simulink model "SOLUTION_04_Control_PID_and_HBridge"  (R2026b)
settings: Solver=ode15s  StopTime=10  MaxStep=0.01  AbsTol=1e-3  EnableMultiTasking=on
undefined symbols (not defined in the file or in its folder): my_DC_moto_OBJ, my_HBridge_OBJ, my_LINK_OBJ, X, Y, Z
libraries: fl_lib x9, sm_lib x8, nesl_utility x4, ee_lib x3, slpidlib x1, simulink x1
settings Model: Creator=bhorton  LastModifiedBy=bhorton
settings SolverCC: AutoScaleAbsTol=off
settings DataIOCC: LimitDataPoints=on  MaxDataPoints=10000
settings OptimizationCC: LifeSpan=inf  ReuseModelBlockBuffer=off
settings DebuggingCC: AllowSymbolicDim=off  ArithmeticOperatorsInVariantConditions=warning  SFExecutionAtInitializationDiag=none  SFNoUnconditionalDefaultTransitionDiag=warning  SFUnexpectedBacktrackingDiag=warning  SubsystemReferenceDiagnosticForUnitTest=warning
settings SFSimCC: CustomCodeUndefinedFunction=UseInterfaceOnly  SimUseLocalCustomCode=off
settings RTWCC: DLArmComputeVersion=19.05  RTWUseLocalCustomCode=off
settings CodeAppCC: StateflowObjectComments=on
settings GRTTargetCC: TargetLangStandard=C89/C90 (ANSI)
settings ConfigComp: CovExternalEMLEnable=off  CovSFcnEnable=off  CovSaveCumulativeToWorkspaceVar=on  CovSaveSingleToWorkspaceVar=on
settings SimscapeCC: SimscapeLogType=all  SimscapeUseEnergyAccounting=off
settings ExplorerConfigSet: InternalSimMechanicsExplorerSettings=|
  | <ExplorerConfiguration>
  | 
  |   <canonicalview>default</canonicalview>
  | 
  |   <TilePanel>
  |     <TileInfo>
  |       <Tiles Columns="2" Count="3" Height="706" Rows="2" Width="1078">
  |         <Row Weight="0.500709"/>
  |         <Row Weight="0.499291"/>
  |         <Column Weight="0.500464"/>
  |         <Column Weight="0.499536"/>
  |         <Tile Height="2" Width="1" X="0" Y="0"/>
  |         <Tile Height="1" Width="1" X="1" Y="0"/>
  |         <Tile Height="1" Width="1" X="1" Y="1"/>
  |       </Tiles>
  |     </TileInfo>
  |     <SceneInfo>
  |       <SceneViewer>
  |         <IsThisViewStd>
  |           <IsStandardView>off</IsStandardView>
  |           <StandardViewName>Front</StandardViewName>
  |         </IsThisViewStd>
  |         <BGColor>
  |           <R>1</R>
  |           <G>1</G>
  |           <B>1</B>
  |           <A>1</A>
  |         </BGColor>
  |         <Camera>
  |           <DoPerspective>off</DoPerspective>
  |           <Position>
  |             <X>0.74892143739918005</X>
  |             <Y>-0.62784979879609726</Y>
  |             <Z>0.69336876380477952</Z>
  |           </Position>
  |           <Center>
  |             <X>0.053221437399180033</X>
  |             <Y>0.067850201203902699</Y>
  |             <Z>-0.0023312361952205086</Z>
  |           </Center>
  |           <Up>
  |             <X>-0.40824829046386307</X>
  |             <Y>0.40824829046386307</Y>
  |             <Z>0.81649658092772615</Z>
  |           </Up>
  |           <XLim>0.18530968569291589</XLim>
  |           <YLim>0.18530968569291589</YLim>
  |           <ViewLimDist>0.01</ViewLimDist>
  |         </Camera>
  |       </SceneViewer>
  |       <SceneViewer>
  |         <IsThisViewStd>
  |           <IsStandardView>off</IsStandardView>
  |           <StandardViewName>Front</StandardViewName>
  |         </IsThisViewStd>
  |         <BGColor>
  |           <R>1</R>
  |           <G>1</G>
  |           <B>1</B>
  |           <A>1</A>
  |         </BGColor>
  |         <Camera>
  |           <DoPerspective>off</DoPerspective>
  |           <Position>
  |             <X>0.024441165727511753</X>
  |             <Y>0.15035032949724758</Y>
  |             <Z>1.8651286729311369</Z>
  |           </Position>
  |           <Center>
  |             <X>0.024441165727511753</X>
  |             <Y>0.15035032949724758</Y>
  |             <Z>0.14374999981373549</Z>
  |           </Center>
  |           <Up>
  |             <X>-1</X>
  |             <Y>-1.8735013540549517e-16</Y>
  |             <Z>0</Z>
  |           </Up>
  |           <XLim>0.15951004814416869</XLim>
  |           <YLim>0.15951004814416869</YLim>
  |           <ViewLimDist>0.01</ViewLimDist>
  |         </Camera>
  |       </SceneViewer>
  |       <SceneViewer>
  |         <IsThisViewStd>
  |           <IsStandardView>off</IsStandardView>
  |           <StandardViewName>Front</StandardViewName>
  |         </IsThisViewStd>
  |         <BGColor>
  |           <R>1</R>
  |           <G>1</G>
  |           <B>1</B>
  |           <A>1</A>
  |         </BGColor>
  |         <Camera>
  |           <DoPerspective>off</DoPerspective>
  |           <Position>
  |             <X>1.4204228299283366</X>
  |             <Y>0.16790494784880997</Y>
  |             <Z>-0.11689190590831854</Z>
  |           </Position>
  |           <Center>
  |             <X>0.096938775434177712</X>
  |             <Y>0.16790494784880997</Y>
  |             <Z>-0.11689190590831854</Z>
  |           </Center>
  |           <Up>
  |             <X>0</X>
  |             <Y>0</Y>
  |             <Z>1</Z>
  |           </Up>
  |           <XLim>0.20515932592869371</XLim>
  |           <YLim>0.20515932592869371</YLim>
  |           <ViewLimDist>0.01</ViewLimDist>
  |         </Camera>
  |       </SceneViewer>
  |     </SceneInfo>
  |   </TilePanel>
  | 
  |   <MechEditorPanel>
  |     <GfxPanelCameraMap/>
  |     <Cameras/>
  |     <VideoCreator>
  |       <IncludeTiles>All</IncludeTiles>
  |       <IncludeTime>on</IncludeTime>
  |       <IncludeWorldFrame>off</IncludeWorldFrame>
  |       <PlaybackSpeedRatio>1</PlaybackSpeedRatio>
  |       <FrameRate>30</FrameRate>
  |       <FrameSize>auto</FrameSize>
  |       <VideoFormat>UncompressedAVI</VideoFormat>
  |     </VideoCreator>
  |   </MechEditorPanel>
  | 
  |   <PlaybackSettings>
  |     <PlaybackSpeedFactor>1</PlaybackSpeedFactor>
  |   </PlaybackSettings>
  | 
  | </ExplorerConfiguration>

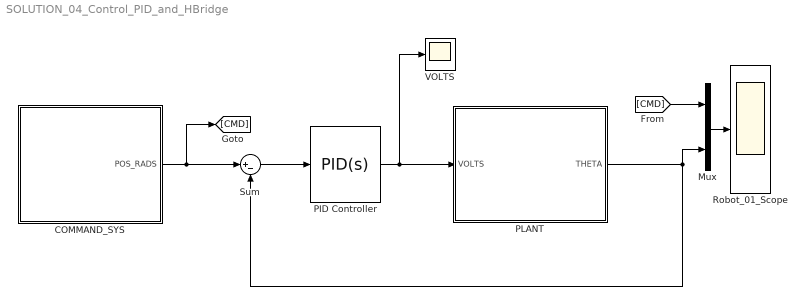
== system SOLUTION_04_Control_PID_and_HBridge ==
  COMMAND_SYS : Subsystem
  Mux : Mux  Inputs=2
  PID Controller : slpidlib/PID Controller  Controller=PID  Form=Parallel  TimeDomain=Continuous-time  UseExternalTs=off  SampleTime=-1  IntegratorMethod=Forward Euler  FilterMethod=Forward Euler  ControllerParametersSource=internal  P=21.8439839664318  I=71.2671260044186  UseKiTs=off  D=1.50425908128224  UseExternalDerivativeSource=off  N=168.946400688862  UseFilter=on  TunerSelectOption=Transfer Function Based (PID Tuner App)  InitialConditionSource=internal  InitialConditionForIntegrator=0  InitialConditionForFilter=0  DifferentiatorICPrevScaledInput=0  ExternalReset=none  TrackingMode=off  Kt=1  LimitOutput=off  SatLimitsSource=internal  UpperSaturationLimit=inf  LowerSaturationLimit=-inf  LinearizeAsGain=on  AntiWindupMode=none  Kb=1  LimitIntegrator=off  UpperIntegratorSaturationLimit=inf  LowerIntegratorSaturationLimit=-inf  POutMin=[]  POutMax=[]  IOutMin=[]  IOutMax=[]  DOutMin=[]  DOutMax=[]  NOutMin=[]  NOutMax=[]  SumOutMin=[]  SumOutMax=[]  SaturationOutMin=[]  SaturationOutMax=[]  PParamMin=[]  PParamMax=[]  IParamMin=[]  IParamMax=[]  DParamMin=[]  DParamMax=[]  NParamMin=[]  NParamMax=[]  KbParamMin=[]  KbParamMax=[]  KtParamMin=[]  KtParamMax=[]  KbOutMin=[]  KbOutMax=[]  KtOutMin=[]  KtOutMax=[]  IntegratorOutMin=[]  IntegratorOutMax=[]  FilterOutMin=[]  FilterOutMax=[]  SumI1OutMin=[]  SumI1OutMax=[]  SumI2OutMin=[]  SumI2OutMax=[]  SumI3OutMin=[]  SumI3OutMax=[]  SumI4OutMin=[]  SumI4OutMax=[]  SumDOutMin=[]  SumDOutMax=[]  DifferentiatorOutMin=[]  DifferentiatorOutMax=[]  FilterDiffOutCoefMin=[]  FilterDiffOutCoefMax=[]  ReciprocalOutMin=[]  ReciprocalOutMax=[]  SumDenOutMin=[]  SumDenOutMax=[]  SumNumOutMin=[]  SumNumOutMax=[]  DivideOutMin=[]  DivideOutMax=[]  UdiffTsProdOutMin=[]  UdiffTsProdOutMax=[]  NTsProdOutMin=[]  NTsProdOutMax=[]  UintegralTsProdOutMin=[]  UintegralTsProdOutMax=[]  UngainTsProdOutMin=[]  UngainTsProdOutMax=[]  ClampingZeroOutDataTypeStr=Inherit: Inherit via back propagation  ClampingZeroOutMin=[]  ClampingZeroOutMax=[]  FilterDenConstantOutDataTypeStr=Inherit: Inherit via back propagation  FilterDenConstantOutMin=[]  FilterDenConstantOutMax=[]  PCopyOutDataTypeStr=Inherit: Inherit via back propagation  PCopyOutMin=[]  PCopyOutMax=[]  NCopyOutDataTypeStr=Inherit: Inherit via back propagation  NCopyOutMin=[]  NCopyOutMax=[]  IntegratorContinuousStateAttributes=''  IntegratorStateMustResolveToSignalObject=off  IntegratorRTWStateStorageClass=Auto  FilterContinuousStateAttributes=''  FilterStateMustResolveToSignalObject=off  FilterRTWStateStorageClass=Auto  ParallelPVariant=InternalParameters  IdealPVariant=Disabled  IVariant=InternalParameters  DVariant=InternalParameters  IntegratorVariant=Continuous  SatVariant=Disabled  AWVariant=Passthrough  PCopyVariant=Disabled  TRVariant=Disabled  FdbkBlocksVariant=Forward  IdealPFdbkVariant=Disabled  SatFdbkVariant=Disabled  DerivativeFilterVariant=ContFilter  NVariant=InternalParameters  NCopyVariant=Disabled  FilterICVariant=InternalICsFilter  IntegratorICVariant=InternalICs  ExternalResetVariant=Disabled  TRSumVariant=Passthrough  SumFdbkVariant=Disabled  SumVariant=Sum_PID  TsampFilterVariant=InternalTs  TsampNgainVariant=Passthrough  TsampIntegralVariant=Disabled_SignalSpec  ExternalSaturationOutDataTypeStr=Inherit: Same as second input  DerivativeSourceVariant=ErrorSignal  PreIntVariant=InternalPreInt
  PLANT : Subsystem
  Robot_01_Scope : Scope
      settings: ActiveDisplayYMinimum=-0.1366602346180848  ActiveDisplayYMaximum=0.954029318573031
  Sum : Sum  Inputs=|+-
  VOLTS : Scope
      settings: ActiveDisplayYMinimum=-3.0831786783905404  ActiveDisplayYMaximum=21.688685222638515  DataLoggingVariableName=ScopeData2
  wires:
  Sum/1 -> PID Controller/1
  PID Controller/1 -> PLANT/1(VOLTS), VOLTS/1
  [CMD] -> Mux/1
  Mux/1 -> Robot_01_Scope/1
  PLANT/1(THETA) -> Sum/2, Mux/2
  COMMAND_SYS/1(POS_RADS) -> [CMD], Sum/1

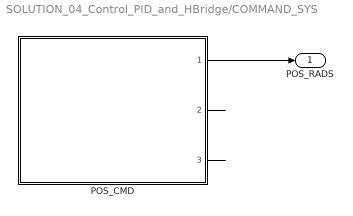
== system SOLUTION_04_Control_PID_and_HBridge/COMMAND_SYS ==
  POS_CMD : Subsystem  ReferencedSubsystem=COMPONENT_POS_CMD
  POS_RADS : Outport
  wires:
  POS_CMD/1 -> POS_RADS/1
  POS_CMD/2 -> ?
  POS_CMD/3 -> ?

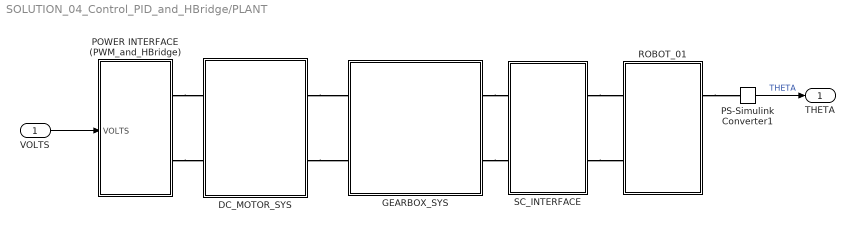
== system SOLUTION_04_Control_PID_and_HBridge/PLANT ==
  VOLTS : Inport
  DC_MOTOR_SYS : Subsystem
  GEARBOX_SYS : Subsystem
  POWER INTERFACE (PWM_and_HBridge) : Subsystem
  PS-Simulink Converter1 : nesl_utility/PS-Simulink Converter  PhysicalDomain=network_engine_domain  SubClassName=ps_output  LeftPortType=input  RightPortType=output  PseudoPeriodic=off  Frequencies=[]  VectorFormat=inherit  Unit=rad  AffineConversion=off
      settings: AttributesFormatString=UNITS= (%<Unit>)
  ROBOT_01 : Subsystem
  SC_INTERFACE : Subsystem
  THETA : Outport
  wires:
  VOLTS/1 -> POWER INTERFACE (PWM_and_HBridge)/1(VOLTS)
  PS-Simulink Converter1/1 -> THETA/1  "THETA"
  connections:
  DC_MOTOR_SYS/RConn1 -- GEARBOX_SYS/LConn1
  SC_INTERFACE/RConn2 -- ROBOT_01/LConn2
  POWER INTERFACE (PWM_and_HBridge)/RConn2 -- DC_MOTOR_SYS/LConn2
  POWER INTERFACE (PWM_and_HBridge)/RConn1 -- DC_MOTOR_SYS/LConn1
  GEARBOX_SYS/RConn2 -- SC_INTERFACE/LConn2
  GEARBOX_SYS/RConn1 -- SC_INTERFACE/LConn1
  SC_INTERFACE/RConn1 -- ROBOT_01/LConn1
  ROBOT_01/RConn1 -- PS-Simulink Converter1/LConn1
  DC_MOTOR_SYS/RConn2 -- GEARBOX_SYS/LConn2

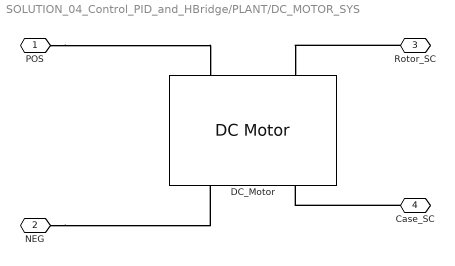
== system SOLUTION_04_Control_PID_and_HBridge/PLANT/DC_MOTOR_SYS ==
  DC_Motor : ee_lib/Electromechanical/Brushed Motors/DC Motor  field_option=ee.enum.field_option.pm  Rf=100 Ohm  Lf=1 H  Laf=0.15 H  If0=0 A  parameterization=ee.enum.dcparam_option.circuit_param  Ra=my_DC_moto_OBJ.arm_R Ohm  La=my_DC_moto_OBJ.arm_L H  emf_or_torque=ee.enum.emf_or_torque.ki  Kv=0.072e-3 V/rpm  Ki=my_DC_moto_OBJ.K_t N*m/A  T_stall=0.24e-3 N*m  w_max=19100 rpm  w_rated=15000 rpm  P_rated=0.08 W  V_rated=1.5 V  lam_param=ee.enum.lam_param.damping  i_noload=0 A  V_i_noload=1.5 V  J=my_DC_moto_OBJ.rotor_I kg*m^2  lam=my_DC_moto_OBJ.rotor_damp N*m*s/rad  speed0=0 rpm  alpha=3.93e-3 1/K  Tmeas=25 degC  thermal_mass=100 J/K  initial_temperature=25 degC
  POS : PMIOPort  Side=Left
  NEG : PMIOPort  Port=2  Side=Left
  Rotor_SC : PMIOPort  Port=3  Side=Right
  Case_SC : PMIOPort  Port=4  Side=Right
  connections:
  NEG/RConn1 -- DC_Motor/RConn1
  POS/RConn1 -- DC_Motor/LConn1
  Rotor_SC/RConn1 -- DC_Motor/LConn2
  Case_SC/RConn1 -- DC_Motor/RConn2

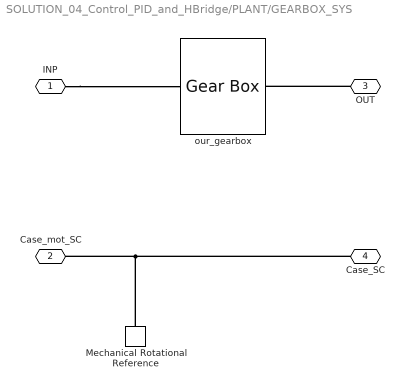
== system SOLUTION_04_Control_PID_and_HBridge/PLANT/GEARBOX_SYS ==
  Mechanical Rotational Reference : fl_lib/Mechanical/Rotational Elements/Mechanical Rotational Reference
  our_gearbox : fl_lib/Mechanical/Mechanisms/Gear Box  ratio=my_gbox_OBJ.N_gear  t_in_specify=off  t_in_priority=None  t_in=0 N*m  t_in_nominal_specify=off  t_in_nominal_value=1  t_in_nominal_unit=N*m  t_out_specify=off  t_out_priority=None  t_out=0 N*m  t_out_nominal_specify=off  t_out_nominal_value=1  t_out_nominal_unit=N*m
      settings: AttributesFormatString=N = w_IN / w_OUT = %<ratio>
  INP : PMIOPort  Side=Left
  Case_mot_SC : PMIOPort  Port=2  Side=Left
  OUT : PMIOPort  Port=3  Side=Right
  Case_SC : PMIOPort  Port=4  Side=Right
  connections:
  Mechanical Rotational Reference/LConn1 -- Case_mot_SC/RConn1 -- Case_SC/RConn1
  INP/RConn1 -- our_gearbox/LConn1
  OUT/RConn1 -- our_gearbox/RConn1

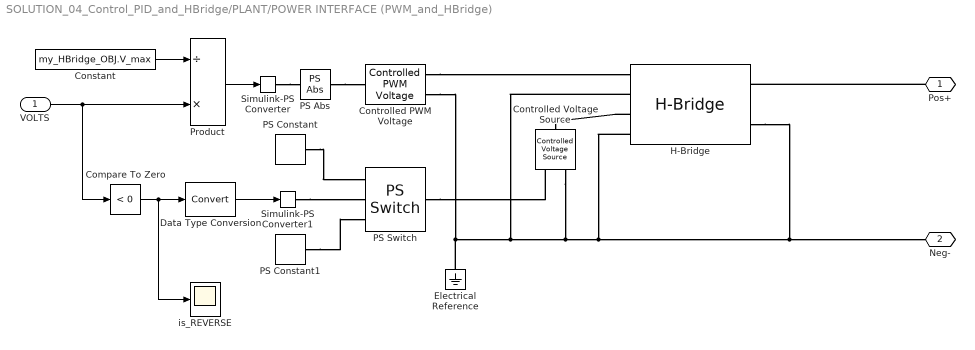
== system SOLUTION_04_Control_PID_and_HBridge/PLANT/POWER INTERFACE (PWM_and_HBridge) ==
  VOLTS : Inport
  Compare To Zero : simulink/Logic and Bit Operations/Compare To Zero  relop=<  OutDataTypeStr=uint8
  Constant : Constant  Value=my_HBridge_OBJ.V_max
  Controlled PWM Voltage : ee_lib/Integrated Circuits/Controlled PWM Voltage  F=80 kHz  TD=0 s  pulse_width_offset=0 s  pulse_min=0 s  pwm_or_av=ee.enum.pwm_or_av.averaged  event_type=ee.enum.ic.event.asynchronous  sample_time=1e-6 s  Vmin=0 V  Vmax=24 V  Vm=my_HBridge_OBJ.V_max V  u_min=0  u_max=1
  Controlled Voltage Source : fl_lib/Electrical/Electrical Sources/Controlled Voltage Source
  Data Type Conversion : DataTypeConversion  SaturateOnIntegerOverflow=off  RndMeth=Floor
  Electrical Reference : fl_lib/Electrical/Electrical Elements/Electrical Reference
  H-Bridge : ee_lib/Semiconductors & Converters/Converters/H-Bridge  supply_ports=ee.enum.supply_ports.hidesupply  pwm_or_av=ee.enum.pwm_or_av.averaged  discontinuous=ee.enum.current_profile.continuous  freewheeling_mode=ee.enum.converters.freewheeling_mode.one_switch_one_diode  Rload=10 Ohm  Lload=1e-5 H  F=10 kHz  regenerative_braking_mode=ee.enum.converters.regenerative_braking_mode.always_enabled  Venable=0.1 V  Vmax=my_HBridge_OBJ.V_max V  Vreverse=2.5 V  Vbrake=2.5 V  Vm=my_HBridge_OBJ.V_max V  Ron=my_HBridge_OBJ.R Ohm  Don=my_HBridge_OBJ.R_diode Ohm  Goff=1e-6 S  Tmeas=298.15 K  Ron2=0.1 Ohm  Don2=0.05 Ohm  Tmeas2=398.15 K  thermal_mass=100 J/K  initial_temperature=298.15 K
  PS Abs : fl_lib/Physical Signals/Nonlinear Operators/PS Abs  ZeroCross=true
  PS Constant : fl_lib/Physical Signals/Sources/PS Constant  constant=5 V
  PS Constant1 : fl_lib/Physical Signals/Sources/PS Constant  constant=0 V
  PS Switch : fl_lib/Physical Signals/Nonlinear Operators/PS Switch  Threshold=0.5  ZeroCross=true
  Product : Product  Inputs=/*
  Simulink-PS Converter : nesl_utility/Simulink-PS Converter  PhysicalDomain=network_engine_domain  SubClassName=ps_input  LeftPortType=input  RightPortType=output  PseudoPeriodic=off  Frequencies=[]  NoiseDistribution=none  NoiseParameters=[]  Unit=1  AffineConversion=off  FilteringAndDerivatives=provide  SimscapeFilterOrder=1  InputFilterTimeConstant=0.001  UdotUserProvided=0
  Simulink-PS Converter1 : nesl_utility/Simulink-PS Converter  PhysicalDomain=network_engine_domain  SubClassName=ps_input  LeftPortType=input  RightPortType=output  PseudoPeriodic=off  Frequencies=[]  NoiseDistribution=none  NoiseParameters=[]  Unit=1  AffineConversion=off  FilteringAndDerivatives=provide  SimscapeFilterOrder=1  InputFilterTimeConstant=0.001  UdotUserProvided=0
  is_REVERSE : Scope
      settings: ActiveDisplayYMinimum=-0.21102162286492421  ActiveDisplayYMaximum=1.2157883377749992  DataLoggingVariableName=ScopeData2
  Pos+ : PMIOPort  Side=Right
  Neg- : PMIOPort  Port=2  Side=Right
  wires:
  VOLTS/1 -> Product/2, Compare To Zero/1
  Data Type Conversion/1 -> Simulink-PS Converter1/1
  Compare To Zero/1 -> is_REVERSE/1, Data Type Conversion/1
  Product/1 -> Simulink-PS Converter/1
  Constant/1 -> Product/1
  connections:
  Pos+/RConn1 -- H-Bridge/RConn1
  Controlled PWM Voltage/RConn1 -- H-Bridge/LConn1
  Controlled PWM Voltage/RConn2 -- Electrical Reference/LConn1 -- H-Bridge/LConn2 -- Controlled Voltage Source/RConn2 -- H-Bridge/LConn4 -- H-Bridge/RConn2 -- Neg-/RConn1
  PS Switch/RConn1 -- Controlled Voltage Source/RConn1
  PS Abs/RConn1 -- Controlled PWM Voltage/LConn1
  PS Constant/RConn1 -- PS Switch/LConn1
  PS Constant1/RConn1 -- PS Switch/LConn3
  Simulink-PS Converter/RConn1 -- PS Abs/LConn1
  H-Bridge/LConn3 -- Controlled Voltage Source/LConn1
  Simulink-PS Converter1/RConn1 -- PS Switch/LConn2

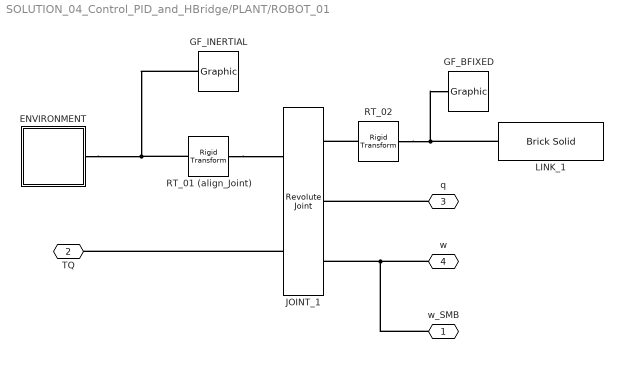
== system SOLUTION_04_Control_PID_and_HBridge/PLANT/ROBOT_01 ==
  ENVIRONMENT : Subsystem
  GF_BFIXED : sm_lib/Body Elements/Graphic  GraphicType=Marker  MarkerShape=Frame  MarkerSize=50  GraphicVisPropType=SimpleVisualProperties  GraphicDiffuseColor=[0.6667 0.6667 1]  GraphicOpacity=1  GraphicSpecularColor=[0.5 0.5 0.5 1.0]  GraphicAmbientColor=[0.15 0.15 0.15 1.0]  GraphicEmissiveColor=[0.0 0.0 0.0 1.0]  GraphicShininess=75
  GF_INERTIAL : sm_lib/Body Elements/Graphic  GraphicType=Marker  MarkerShape=Frame  MarkerSize=55  GraphicVisPropType=SimpleVisualProperties  GraphicDiffuseColor=[1 0 0]  GraphicOpacity=1  GraphicSpecularColor=[0.5 0.5 0.5 1.0]  GraphicAmbientColor=[0.15 0.15 0.15 1.0]  GraphicEmissiveColor=[0.0 0.0 0.0 1.0]  GraphicShininess=75
  JOINT_1 : sm_lib/Joints/Revolute Joint  JointMode=Normal  CompositeWrenchDir=FollowerOnBase  CompositeWrenchFrame=BaseFrame  SenseConstraintForce=off  SenseConstraintTorque=off  SenseTotalForce=off  SenseTotalTorque=off  PositionTargetSpecify=on  PositionTargetPriority=High  PositionTargetValue=my_joint_1_OBJ.theta  PositionTargetValueUnits=rad  VelocityTargetSpecify=on  VelocityTargetPriority=High  VelocityTargetValue=my_joint_1_OBJ.theta_dot  VelocityTargetValueUnits=rad/s  EquilibriumPosition=0  EquilibriumPositionUnits=deg  SpringStiffness=0  SpringStiffnessUnits=N*m/deg  DampingCoefficient=my_joint_1_OBJ.Damp  DampingCoefficientUnits=N*m*s/rad  LowerLimitSpecify=off  LowerLimitBound=-90  LowerLimitBoundUnits=deg  LowerLimitStiffness=1e4  LowerLimitStiffnessUnits=N*m/deg  LowerLimitDamping=10  LowerLimitDampingUnits=N*m/(deg/s)  LowerLimitTransitionRegionWidth=0.1  LowerLimitTransitionRegionWidthUnits=deg  UpperLimitSpecify=off  UpperLimitBound=90  UpperLimitBoundUnits=deg  UpperLimitStiffness=1e4  UpperLimitStiffnessUnits=N*m/deg  UpperLimitDamping=10  UpperLimitDampingUnits=N*m/(deg/s)  UpperLimitTransitionRegionWidth=0.1  UpperLimitTransitionRegionWidthUnits=deg  TorqueActuationMode=InputTorque  MotionActuationMode=ComputedMotion  SensePosition=on  SenseVelocity=on  SenseAcceleration=off  SenseTorqueForce=off  SenseLowerLimitTorqueForce=off  SenseUpperLimitTorqueForce=off
  LINK_1 : sm_lib/Body Elements/Brick Solid  BrickDimensions=my_LINK_OBJ.vec_XYZ  BrickDimensionsUnits=m  ExportEntireGeometry=off  InertiaType=CalculateFromGeometry  BasedOnType=Mass  Density=1000  DensityUnits=kg/m^3  Mass=my_LINK_OBJ.Mass  MassUnits=kg  CenterOfMass=[0 0 0]  CenterOfMassUnits=m  MomentsOfInertia=[1 1 1]  MomentsOfInertiaUnits=kg*m^2  ProductsOfInertia=[0 0 0]  ProductsOfInertiaUnits=kg*m^2  GraphicType=FromGeometry  MarkerShape=Sphere  MarkerSize=10  GraphicVisPropType=SimpleVisualProperties  GraphicDiffuseColor=[0 0.6667 1]  GraphicOpacity=1.0  GraphicSpecularColor=[0.5 0.5 0.5 1.0]  GraphicAmbientColor=[0.15 0.15 0.15 1.0]  GraphicEmissiveColor=[0.0 0.0 0.0 1.0]  GraphicShininess=75  DoExposeReferenceFrame=on  SerializedFrames=|
      | <Frames>
      | 
      |   <Frame>
      |     <Id>Frame1</Id>
      |     <Value>
      |       <Name>LEFT</Name>
      |       <Origin>
      |         <Source>GeometricFeature</Source>
      |         <FeatureName>-y surface</FeatureName>
      |       </Origin>
      |       <PrimaryAxis>
      |         <DefinedDirection>+Z</DefinedDirection>
      |         <Source>ReferenceFrame</Source>
      |         <SourceDirection>+Z</SourceDirection>
      |         <FeatureName></FeatureName>
      |       </PrimaryAxis>
      |       <SecondaryAxis>
      |         <DefinedDirection>+X</DefinedDirection>
      |         <Source>ReferenceFrame</Source>
      |         <SourceDirection>+X</SourceDirection>
      |         <FeatureName></FeatureName>
      |       </SecondaryAxis>
      |     </Value>
      |   </Frame>
      | 
      | </Frames>
  RT_01 (align_Joint) : sm_lib/Frames and Transforms/Rigid Transform  RotationMethod=StandardAxis  FollAlignAxisA=+Z  BaseAlignAxisA=+X  FollAlignAxisB=+Y  BaseAlignAxisB=+Y  RotationStandardAxis=+Y  RotationAngle=90  RotationAngleUnits=deg  RotationArbitraryAxis=[0 0 1]  RotationSequenceAxes=FollowerAxes  RotationSequence=XYX  RotationSequenceAngles=[0 0 0]  RotationSequenceAnglesUnits=deg  RotationMatrix=[1 0 0;0 1 0;0 0 1]  Quaternion=[1 0 0 0]  TranslationMethod=None  TranslationCartesianOffset=[0 0 0]  TranslationCartesianOffsetUnits=m  TranslationStandardAxis=+Z  TranslationStandardOffset=0  TranslationStandardOffsetUnits=m  TranslationROffset=0  TranslationROffsetUnits=m  TranslationThetaOffset=0  TranslationThetaOffsetUnits=deg  TranslationZOffset=0  TranslationZOffsetUnits=m
  RT_02 : sm_lib/Frames and Transforms/Rigid Transform  RotationMethod=StandardAxis  FollAlignAxisA=+X  BaseAlignAxisA=+Z  FollAlignAxisB=+Y  BaseAlignAxisB=+Y  RotationStandardAxis=+Y  RotationAngle=-90  RotationAngleUnits=deg  RotationArbitraryAxis=[0 0 1]  RotationSequenceAxes=FollowerAxes  RotationSequence=XYX  RotationSequenceAngles=[0 0 0]  RotationSequenceAnglesUnits=deg  RotationMatrix=[1 0 0;0 1 0;0 0 1]  Quaternion=[1 0 0 0]  TranslationMethod=None  TranslationCartesianOffset=[0 0 0]  TranslationCartesianOffsetUnits=m  TranslationStandardAxis=+Z  TranslationStandardOffset=0  TranslationStandardOffsetUnits=m  TranslationROffset=0  TranslationROffsetUnits=m  TranslationThetaOffset=0  TranslationThetaOffsetUnits=deg  TranslationZOffset=0  TranslationZOffsetUnits=m
  w_SMB : PMIOPort  Side=Left
  TQ : PMIOPort  Port=2  Side=Left
  q : PMIOPort  Port=3  Side=Right
  w : PMIOPort  Port=4  Side=Right
  connections:
  RT_02/RConn1 -- LINK_1/LConn1 -- GF_BFIXED/RConn1
  GF_INERTIAL/RConn1 -- ENVIRONMENT/RConn1 -- RT_01 (align_Joint)/LConn1
  RT_01 (align_Joint)/RConn1 -- JOINT_1/LConn1
  RT_02/LConn1 -- JOINT_1/RConn1
  q/RConn1 -- JOINT_1/RConn2
  w/RConn1 -- w_SMB/RConn1 -- JOINT_1/RConn3
  JOINT_1/LConn2 -- TQ/RConn1

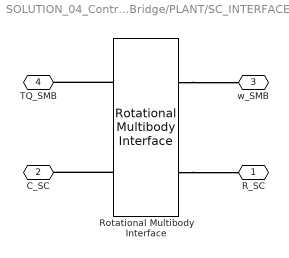
== system SOLUTION_04_Control_PID_and_HBridge/PLANT/SC_INTERFACE ==
  Rotational Multibody Interface : fl_lib/Mechanical/Multibody Interfaces/Rotational Multibody Interface
  R_SC : PMIOPort  Side=Left
  C_SC : PMIOPort  Port=2  Side=Left
  w_SMB : PMIOPort  Port=3  Side=Right
  TQ_SMB : PMIOPort  Port=4  Side=Right
  connections:
  Rotational Multibody Interface/LConn1 -- TQ_SMB/RConn1
  Rotational Multibody Interface/LConn2 -- C_SC/RConn1
  Rotational Multibody Interface/RConn1 -- w_SMB/RConn1
  Rotational Multibody Interface/RConn2 -- R_SC/RConn1

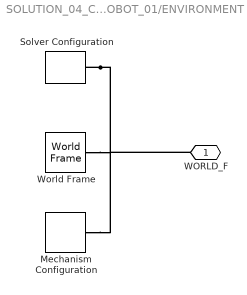
== system SOLUTION_04_Control_PID_and_HBridge/PLANT/ROBOT_01/ENVIRONMENT ==
  Mechanism Configuration : sm_lib/Utilities/Mechanism Configuration  UniformGravity=Constant  GravityVector=gravity_vec  GravityVectorUnits=m/s^2  LinearizationDelta=0.001  JointModeTransitionNonlinearIterations=2
  Solver Configuration : nesl_utility/Solver Configuration  PhysicalDomain=network_engine_domain  SubClassName=solver  LeftPortType=input  RightPortType=generic  Tones=[]  Harmonics=[]  SimulateNoise=off  Profile=off  UseLocalSampling=off  EnableSwitchedLinearOptims=on  FrequencyDomain=off  UseCCode=off  RelTol=0.001  AbsTol=1e-06  MinStep=1e-09  ToWorkspace=off  RevertToSquareIcSolve=off  NumHomotopyIterations=100  PhasorMode=off  PhasorModeNumHarmonics=1  ConsistencySolver=NEWTON_XTOL_AFTER_FTOL  CanonicalOrdering=UNORDERED  OptimizeIntermediates=UNOPTIMIZED  MulticoreSolverChoice=BACKWARD_EULER  IndexReductionMethod=DerivativeReplacement  DoDC=off  ResidualTolerance=1e-09  ConsistencyTolSource=GLOBAL  ConsistencyAbsTol=0.001  ConsistencyRelTol=0.001  ConsistencyTolFactor=0.001  UseLocalSolver=off  LocalSolverChoice=NE_BACKWARD_EULER_ADVANCER  ResolveIndetEquations=on  FunctionEvalNumThread=1  LocalSolverSampleTime=0.001  DoFixedCost=off  MaxNonlinIter=3  MaxModeIter=2  ComputeImpulses=off  ImpulseIterations=2  LinearAlgebra=Sparse  LinearAlgebraNumThread=0  EquationFormulation=NE_TIME_EF  DelaysMemoryBudget=1024  AutomaticFiltering=on  FilteringTimeConstant=0.001  PartitionStorageMethod=AS_NEEDED  PartitionMemoryBudget=1024  PartitionMethod=FAST  MultibodyUseLocalSolver=off  MultibodyLocalSolverChoice=ODE1  MultibodyLocalSolverSampleTime=0.001
  World Frame : sm_lib/Frames and Transforms/World Frame
  WORLD_F : PMIOPort  Side=Right
  connections:
  Solver Configuration/RConn1 -- World Frame/RConn1 -- Mechanism Configuration/RConn1 -- WORLD_F/RConn1
